simulink model "Radial_Grid"  (R2024a)
settings: Solver=VariableStepAuto  StartTime=0.0  StopTime=1  RelTol=1e-3
undefined symbols (not defined in the file): D1, Delta
libraries: spsThreePhaseBreakerLib x8, spsGroundLib x7, spsThreePhaseParallelRLCLoadLib x7, spsThreePhaseVIMeasurementLib x5, eeRmsMeasurement x2, spsDistributedParametersLineLib x1, spsPLL3phLib x1, spsThreePhaseSourceLib x1, spsThreePhaseTransformerInductanceMatrixTypeTwoWindingsLib x1, sps_lib x1
settings Model: Creator=NIHUB  LastModifiedBy=NIHUB

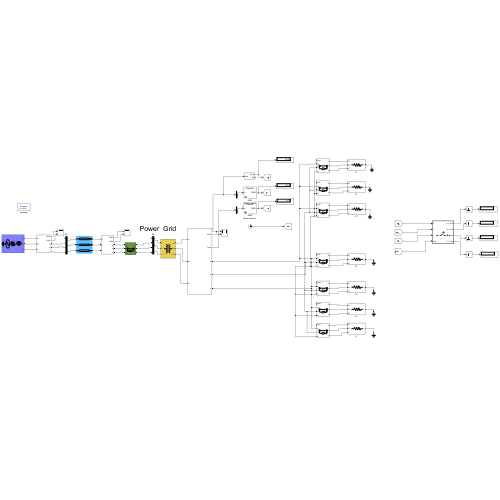
[thumbnail: Simulink's stored preview of the top-level diagram]
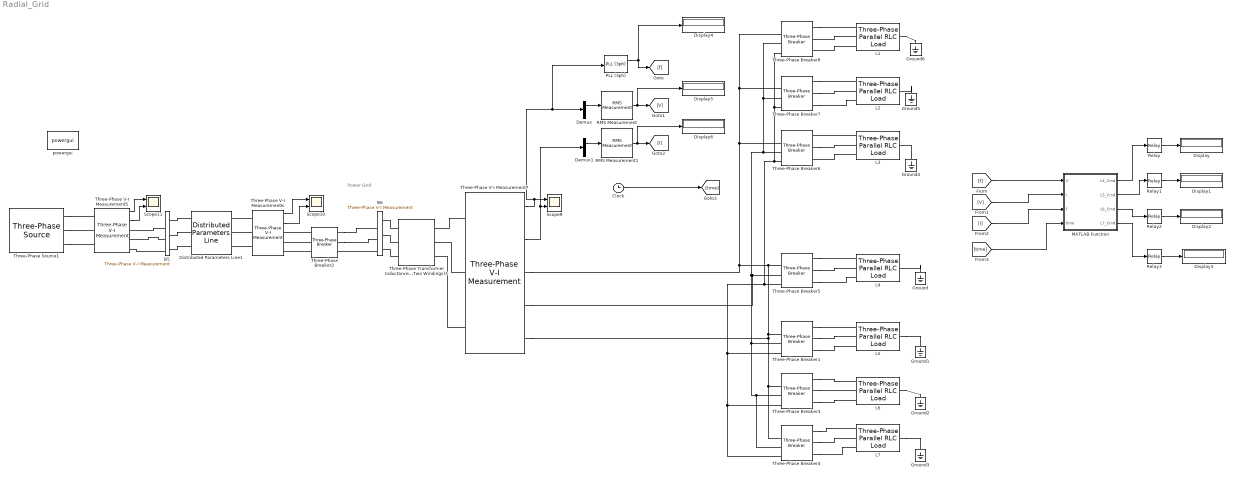
== system Radial_Grid ==
  note: Power Grid
  B5 : spsThreePhaseVIMeasurementLib/Three-Phase V-I Measurement  VoltageMeasurement=phase-to-ground  SetLabelV=off  LabelV=Vabc_B12  Vpu=off  VpuLL=off  CurrentMeasurement=no  SetLabelI=off  LabelI=A1  Ipu=off  Pbase=100e6  Vbase=25e3  OutputType=Magnitude  PhasorSimulation=off  PSBequivalent=0
  B6 : spsThreePhaseVIMeasurementLib/Three-Phase V-I Measurement  VoltageMeasurement=phase-to-phase  SetLabelV=off  LabelV=Vabc_B12  Vpu=off  VpuLL=off  CurrentMeasurement=no  SetLabelI=off  LabelI=A1  Ipu=off  Pbase=100e6  Vbase=440  OutputType=Magnitude  PhasorSimulation=off  PSBequivalent=0
  Clock : Clock
  Demux : Demux  Outputs=3
  Demux1 : Demux  Outputs=3
  Display{,1..6} (7 alike) : Display
  Distributed Parameters Line1 : spsDistributedParametersLineLib/Distributed Parameters Line  Phases=3  Length=100  Frequency=50  Resistance=[0.01273 0.3864]  Inductance="[0.9337e-3  4.1264e-3]"  Capacitance=[12.74e-9 7.751e-9]  x1=[-0.0006 -5.69435652062801e-12 3198.12006317178 -10428.926964129;-0.00055 -5.76202165425784e-12 3395.1058429697 -10367.660250018;-0.0005 -5.82763956903046e-12 3590.88535782781 -10302.709955587;-0.00045 -5.8911869512132e-12 3785.38904821671 -10234.0991573664;-0.0004 -5.95264122272375e-12 3978.54780790135 -10161.852232446;-0.00035 -6.01198054915207e-12 4170.29300849417 -10085.9948498143;-0.0003 -6.06918384751803e-12 4360.55652383841 -10006.5539612381;-0.00025 -6.1242307937621e-12 4549.27075421304 -9923.55779168682;-0.0002 -6.1771018299664e-12 4736.36865035058 -9837.03582930438;-0.00015 -6.22777817130351e-12 4921.78373725944 -9747.018814932;-0.0001 -6.27624181271066e-12 5105.4501378421 -9653.53873118626;-5e-05 -6.32247553528681e-12 5287.30259630099 -9556.62879109579]  x2=[-0.0006 9.88072191954148e-12 2341.94542948647 -8036.57356519092;-0.00055 3.91022286306686e-12 2519.49823419962 -8019.58597186587;-0.0005 -2.06166547697203e-12 2696.15587318705 -7999.74905783124;-0.00045 -8.03282131708381e-12 2871.8555808308 -7977.0698710481;-0.0004 -1.40011231340308e-11 3046.53493186135 -7951.55646932354;-0.00035 -1.99644504185964e-11 3220.13186353705 -7923.2179174477;-0.0003 -2.59206844289913e-11 3392.58469769468 -7892.06428397313;-0.00025 -3.18677089436329e-11 3563.83216266341 -7858.10663763746;-0.0002 -3.78034110130288e-11 3733.81341503435 -7821.35704343074;-0.00015 -4.37256817104971e-11 3902.46806127792 -7781.82855830881;-0.0001 -4.96324168814587e-11 4069.73617920138 -7739.5352265542;-5e-05 -5.55215178910329e-11 4235.5583392389 -7694.4920747863]  x3=[-0.0006 1.90091766669321e-12 37.8763934062412 29.3478799697958;-0.00055 1.89376898505282e-12 38.1331821574926 30.7493103327158;-0.0005 1.88594745630945e-12 38.376422370699 32.139815612091;-0.00045 1.87745585941501e-12 38.606027623771 33.5189017680168;-0.0004 1.86829721139346e-12 38.8219163390555 34.8860788177486;-0.00035 1.85847476626881e-12 39.0240118123198 36.2408610097907;-0.0003 1.84799201390905e-12 39.2122422400046 37.5827669964811;-0.00025 1.83685267878618e-12 39.3865407447353 38.9113200050124;-0.0002 1.82506071865293e-12 39.546845399083 40.2260480068268;-0.00015 1.81262032313659e-12 39.6930992475674 41.5264838853255;-0.0001 1.79953591225044e-12 39.8252503268925 42.8121656018329;-5e-05 1.78581213482337e-12 39.9432516844091 44.0826363597572]  x4=[-0.0006 -1.86563145591836e-12 -22.2642144665342 -98.2708522257449;-0.00055 -1.86603152740087e-12 -21.1164830183401 -99.4675733684154;-0.0005 -1.86576860676702e-12 -19.9612489842783 -100.628954155895;-0.00045 -1.86484278743127e-12 -18.7989228135002 -101.754581955119;-0.0004 -1.86325439833281e-12 -17.6299174749598 -102.844056835891;-0.00035 -1.86100400381873e-12 -16.4546483106874 -103.896991712974;-0.0003 -1.85809240344349e-12 -15.2735328882211 -104.913012483619;-0.00025 -1.85452063168482e-12 -14.0869908522462 -105.891758160483;-0.0002 -1.85028995757624e-12 -12.8954437754984 -106.83288099989;-0.00015 -1.84540188425611e-12 -11.6993150089804 -107.736046625375;-0.0001 -1.8398581484336e-12 -10.4990295315473 -108.600934146491;-5e-05 -1.83366071977165e-12 -9.29501379891409 -109.427236272822]  x5=0.000565541566995743  V1=[0 0 0 2.339e-09 6.456e+04 6.456e+04;0 0 0 314.2 314.2 314.2;1.571 1.571 1.571 -0.9334 0.4129 -1.158]  V2=[0 0 0 9.955e-09 6.494e+04 6.494e+04;0 0 0 314.2 314.2 314.2;1.571 1.571 1.571 -1.047 0.4126 -1.158]  I1=[0 0 0 5.638e-11 239 239;0 0 0 314.2 314.2 314.2;1.571 1.571 1.571 -2.312 0.3045 -1.266]  I2=[0 0 0 5.238e-11 239.1 239.1;0 0 0 314.2 314.2 314.2;1.571 1.571 1.571 0.5382 0.4125 -1.158]  nHarmo=2  Measurements=None  Decoupling=off  VsMag0=0  VrMag0=0  VsAngle0=0  VrAngle0=0  IsMag0=0  IrMag0=0  IsAngle0=0  IrAngle0=0
      settings: LibrarySourceBlock=sps_lib/Power Grid Elements/Distributed Parameters Line
  Ground{,1..6} (7 alike) : spsGroundLib/Ground  LConnTagsString=a
  L1 : spsThreePhaseParallelRLCLoadLib/Three-Phase Parallel RLC Load  LConnTagsString=A|B|C  RConnTagsString=N  Configuration=Y (neutral)  NominalVoltage=400  Vabc=[1e3 1e3 1e3]  Vabcp=[1e3 1e3 1e3]  NominalFrequency=50  UnbalancedPower=off  ActivePower=300e3  InductivePower=0  CapacitivePower=0  Pabc=[10e3 9e3 11e3]  QLabc=[100 90 110]  QCabc=[100 90 110]  Pabcp=[10e3 9e3 11e3]  QLabcp=[100 90 110]  QCabcp=[100 90 110]  Measurements=Branch voltages and currents  LoadType=constant PQ
  L2 : spsThreePhaseParallelRLCLoadLib/Three-Phase Parallel RLC Load  LConnTagsString=A|B|C  RConnTagsString=N  Configuration=Y (neutral)  NominalVoltage=400  Vabc=[1e3 1e3 1e3]  Vabcp=[1e3 1e3 1e3]  NominalFrequency=50  UnbalancedPower=off  ActivePower=250e3  InductivePower=0  CapacitivePower=0  Pabc=[10e3 9e3 11e3]  QLabc=[100 90 110]  QCabc=[100 90 110]  Pabcp=[10e3 9e3 11e3]  QLabcp=[100 90 110]  QCabcp=[100 90 110]  Measurements=Branch voltages and currents  LoadType=constant PQ
  L3 : spsThreePhaseParallelRLCLoadLib/Three-Phase Parallel RLC Load  LConnTagsString=A|B|C  RConnTagsString=N  Configuration=Y (neutral)  NominalVoltage=400  Vabc=[1e3 1e3 1e3]  Vabcp=[1e3 1e3 1e3]  NominalFrequency=50  UnbalancedPower=off  ActivePower=200e3  InductivePower=0  CapacitivePower=0  Pabc=[10e3 9e3 11e3]  QLabc=[100 90 110]  QCabc=[100 90 110]  Pabcp=[10e3 9e3 11e3]  QLabcp=[100 90 110]  QCabcp=[100 90 110]  Measurements=Branch voltages and currents  LoadType=constant PQ
  L4 : spsThreePhaseParallelRLCLoadLib/Three-Phase Parallel RLC Load  LConnTagsString=A|B|C  RConnTagsString=N  Configuration=Y (neutral)  NominalVoltage=400  Vabc=[1e3 1e3 1e3]  Vabcp=[1e3 1e3 1e3]  NominalFrequency=50  UnbalancedPower=off  ActivePower=180e3  InductivePower=0  CapacitivePower=0  Pabc=[10e3 9e3 11e3]  QLabc=[100 90 110]  QCabc=[100 90 110]  Pabcp=[10e3 9e3 11e3]  QLabcp=[100 90 110]  QCabcp=[100 90 110]  Measurements=Branch voltages and currents  LoadType=constant PQ
  L5 : spsThreePhaseParallelRLCLoadLib/Three-Phase Parallel RLC Load  LConnTagsString=A|B|C  RConnTagsString=N  Configuration=Y (neutral)  NominalVoltage=400  Vabc=[1e3 1e3 1e3]  Vabcp=[1e3 1e3 1e3]  NominalFrequency=50  UnbalancedPower=off  ActivePower=120e3  InductivePower=0  CapacitivePower=0  Pabc=[10e3 9e3 11e3]  QLabc=[100 90 110]  QCabc=[100 90 110]  Pabcp=[10e3 9e3 11e3]  QLabcp=[100 90 110]  QCabcp=[100 90 110]  Measurements=Branch voltages and currents  LoadType=constant PQ
  L6 : spsThreePhaseParallelRLCLoadLib/Three-Phase Parallel RLC Load  LConnTagsString=A|B|C  RConnTagsString=N  Configuration=Y (neutral)  NominalVoltage=400  Vabc=[1e3 1e3 1e3]  Vabcp=[1e3 1e3 1e3]  NominalFrequency=50  UnbalancedPower=off  ActivePower=100e3  InductivePower=0  CapacitivePower=0  Pabc=[10e3 9e3 11e3]  QLabc=[100 90 110]  QCabc=[100 90 110]  Pabcp=[10e3 9e3 11e3]  QLabcp=[100 90 110]  QCabcp=[100 90 110]  Measurements=Branch voltages and currents  LoadType=constant PQ
  L7 : spsThreePhaseParallelRLCLoadLib/Three-Phase Parallel RLC Load  LConnTagsString=A|B|C  RConnTagsString=N  Configuration=Y (neutral)  NominalVoltage=400  Vabc=[1e3 1e3 1e3]  Vabcp=[1e3 1e3 1e3]  NominalFrequency=50  UnbalancedPower=off  ActivePower=150e3  InductivePower=0  CapacitivePower=0  Pabc=[10e3 9e3 11e3]  QLabc=[100 90 110]  QCabc=[100 90 110]  Pabcp=[10e3 9e3 11e3]  QLabcp=[100 90 110]  QCabcp=[100 90 110]  Measurements=Branch voltages and currents  LoadType=constant PQ
  MATLAB Function : MATLAB Function  TreatAsAtomicUnit=on
  PLL (3ph) : spsPLL3phLib/PLL (3ph)  Fmin=45  Par_Init=[0, 50]  ParK=[180, 3200, 1]  TcD=1e-4  MaxRateChangeFreq=12  FilterCutOffFreq=25  Ts=50e-6  AGC=on
  RMS Measurement : eeRmsMeasurement/RMS Measurement  LabelModeActiveChoice=Total  F=50  SpecifyHarmonics=off  K=[0 1 2]  Ts=50e-6
      settings: LibrarySourceBlock=|
      | ee_sl_lib/Measurements/RMS
      | Measurement
  RMS Measurement1 : eeRmsMeasurement/RMS Measurement  LabelModeActiveChoice=Total  F=50  SpecifyHarmonics=off  K=[0 1 2]  Ts=50e-6
      settings: LibrarySourceBlock=|
      | ee_sl_lib/Measurements/RMS
      | Measurement
  Relay{,1..3} (4 alike) : Relay
  Scope10 : Scope  NumInputPorts=2
  Scope11 : Scope  NumInputPorts=2
  Scope9 : Scope  NumInputPorts=2
  Three-Phase V-I Measurement5 : spsThreePhaseVIMeasurementLib/Three-Phase V-I Measurement  VoltageMeasurement=phase-to-ground  SetLabelV=off  LabelV=Vabc  Vpu=off  VpuLL=off  CurrentMeasurement=yes  SetLabelI=off  LabelI=Iabc  Ipu=off  Pbase=100e6  Vbase=500e3  OutputType=Complex  PhasorSimulation=off  PSBequivalent=0
  Three-Phase V-I Measurement6 : spsThreePhaseVIMeasurementLib/Three-Phase V-I Measurement  VoltageMeasurement=phase-to-ground  SetLabelV=off  LabelV=Vabc  Vpu=off  VpuLL=off  CurrentMeasurement=yes  SetLabelI=off  LabelI=Iabc  Ipu=off  Pbase=100e6  Vbase=500e3  OutputType=Complex  PhasorSimulation=off  PSBequivalent=0
  Three-Phase V-I Measurement7 : spsThreePhaseVIMeasurementLib/Three-Phase V-I Measurement  VoltageMeasurement=phase-to-phase  SetLabelV=off  LabelV=Vabc_b1  Vpu=off  VpuLL=off  CurrentMeasurement=yes  SetLabelI=off  LabelI=Iabc_b1  Ipu=off  Pbase=100e6  Vbase=500e3  OutputType=Complex  PhasorSimulation=off  PSBequivalent=0
  Three-Phase Breaker{1,3..8} (7 alike) : spsThreePhaseBreakerLib/Three-Phase Breaker  InitialState=closed  SwitchA=off  SwitchB=off  SwitchC=off  SwitchTimes="[1/60  5/60]"  External=on  BreakerResistance=0.01  SnubberResistance=1e6  SnubberCapacitance=inf  Measurements=None
  Three-Phase Breaker2 : spsThreePhaseBreakerLib/Three-Phase Breaker  InitialState=closed  SwitchA=off  SwitchB=off  SwitchC=off  SwitchTimes="[1/50  20/50]"  External=off  BreakerResistance=0.001  SnubberResistance=1e6  SnubberCapacitance=inf  Measurements=None
  Three-Phase Source1 : spsThreePhaseSourceLib/Three-Phase Source  InternalConnection=Yg  VoltagePhases=off  Voltage=11000  PhaseAngle=0  Voltage_phases=[25e3 25e3 25e3]/sqrt(3)  PhaseAngles_phases=[0 -120 +120]  Frequency=60  NonIdealSource=on  SpecifyImpedance=on  Resistance=0.8929  Inductance=16.58e-3  ShortCircuitLevel=100e6  BaseVoltage=11000  XRratio=7  BusType=swing  Pref=0  Qref=0  Prefabc=[10e3, 10e3, 10e3]  Qrefabc=[0, 0, 0]  Qmin=-inf  Qmax=inf
  Three-Phase Transformer Inductance Matrix Type (Two Windings)3 : spsThreePhaseTransformerInductanceMatrixTypeTwoWindingsLib/Three-Phase Transformer Inductance Matrix Type (Two Windings)  CoreType=Three-limb or five-limb core  Winding1Connection=Delta (D1)  Winding2Connection=Delta (D1)  AutoTransformer=off  Measurements=None  NominalPower=[100e3 50]  VLLnom=[11000 400]  WindingResistances=[0.01 0.01]  NoLoadIexcPos=2  NoLoadPlossPos=1000  ShortCircuitReactancePos=0.06  ShortCircuitReactancePosAuto=0.06  NoLoadIexcZero=100  NoLoadPlossZero=1500  ShortCircuitReactanceZero=0.03  ShortCircuitReactanceZeroAuto=0.03
      settings: LibrarySourceBlock=|
      | sps_lib/Power Grid Elements/Three-Phase Transformer
      | Inductance Matrix Type
      | (Two Windings)
  powergui : sps_lib/powergui  Priority=1  SimulationMode=Discrete  SampleTime=50e-6  frequency=60  Iterations=50  frequencyindice=0  Pbase=100e6  ErrMax=1e-4  UnitsV=kV  UnitsW=MW  buscounter=0  FunctionMessages=off  echomessages=off  EnableUseOfTLC=off  CurrentSourceSwitches=off  DisableSnubberDevices=off  DisableRonSwitches=off  DisableVfSwitches=off  DisplayEquations=off  AutomaticDiscreteSolvers=off  SolverType=Tustin  Interpol=off  ExternalGateDelay=off  methode=off  Ts=0  x0status=blocks  SPID=off  SwTol=0  HookPort=off  NonlinearTolerance=1e-4  nMaxIteration=100  ContinueOnMaxIteration=off  RestoreLinks=warning  ResistiveCurrentMeasurement=off  Frange=[0:2:500]  Ylog=off  Xlog=on  ShowGrid=off  save=off  variable=ZData  structure=0  ZoomFFT=off  StartTime=0.0  cycles=1  DisplayStyle=1  fundamental=60  FreqAxis=off  MaxFrequency=1000  frequencyindicesteady=1  RmsSteady=1  display=off
  wires:
  [f] -> MATLAB Function/1(V)
  [V] -> MATLAB Function/2(I)
  [I] -> MATLAB Function/3(f)
  [time] -> MATLAB Function/4(time)
  MATLAB Function/1(L4_Cmd) -> Relay/1
  MATLAB Function/2(L5_Cmd) -> Relay1/1
  MATLAB Function/3(L6_Cmd) -> Relay2/1
  MATLAB Function/4(L7_Cmd) -> Relay3/1
  Relay3/1 -> Display3/1
  Relay2/1 -> Display2/1
  Relay1/1 -> Display1/1
  Relay/1 -> Display/1
  Demux1/1 -> RMS Measurement1/1
  RMS Measurement/1 -> Display5/1, [V]
  RMS Measurement1/1 -> Display6/1, [I]
  Three-Phase V-I Measurement6/1 -> Scope10/1
  Three-Phase V-I Measurement5/2 -> Scope11/2
  Three-Phase V-I Measurement5/1 -> Scope11/1
  Three-Phase V-I Measurement7/2 -> Demux1/1, Scope9/2
  Three-Phase V-I Measurement6/2 -> Scope10/2
  Demux/1 -> RMS Measurement/1
  PLL (3ph)/1 -> Display4/1, [f]
  Three-Phase V-I Measurement7/1 -> PLL (3ph)/1, Demux/1, Scope9/1
  Clock/1 -> [time]
  connections:
  Ground/LConn1 -- L4/RConn1
  Ground5/LConn1 -- L2/RConn1
  L1/RConn1 -- Ground6/LConn1
  Ground4/LConn1 -- L3/RConn1
  L5/RConn1 -- Ground1/LConn1
  L6/RConn1 -- Ground2/LConn1
  L7/RConn1 -- Ground3/LConn1
  Three-Phase Breaker1/RConn1 -- L5/LConn1
  Three-Phase Breaker1/RConn2 -- L5/LConn2
  Three-Phase Breaker1/RConn3 -- L5/LConn3
  Three-Phase Breaker3/RConn1 -- L6/LConn1
  Three-Phase Breaker3/RConn2 -- L6/LConn2
  Three-Phase Breaker3/RConn3 -- L6/LConn3
  Three-Phase Breaker4/RConn1 -- L7/LConn1
  Three-Phase Breaker4/RConn2 -- L7/LConn2
  Three-Phase Breaker4/RConn3 -- L7/LConn3
  Three-Phase Breaker5/RConn1 -- L4/LConn1
  Three-Phase Breaker5/RConn2 -- L4/LConn2
  Three-Phase Breaker5/RConn3 -- L4/LConn3
  Three-Phase Breaker5/LConn1 -- Three-Phase Breaker4/LConn1 -- Three-Phase Breaker3/LConn1 -- Three-Phase V-I Measurement7/RConn3 -- Three-Phase Breaker1/LConn1 -- Three-Phase Breaker8/LConn1 -- Three-Phase Breaker7/LConn1 -- Three-Phase Breaker6/LConn1 -- Three-Phase V-I Measurement7/RConn1
  Three-Phase Breaker4/LConn2 -- Three-Phase Breaker3/LConn2 -- Three-Phase Breaker1/LConn2 -- Three-Phase Breaker8/LConn2 -- Three-Phase Breaker7/LConn2 -- Three-Phase Breaker6/LConn2 -- Three-Phase V-I Measurement7/RConn2 -- Three-Phase Breaker5/LConn2
  Three-Phase Breaker1/LConn3 -- Three-Phase Breaker4/LConn3 -- Three-Phase Breaker3/LConn3 -- Three-Phase Breaker8/LConn3 -- Three-Phase Breaker7/LConn3 -- Three-Phase Breaker6/LConn3 -- Three-Phase Breaker5/LConn3
  Three-Phase Breaker8/RConn1 -- L1/LConn1
  L1/LConn2 -- Three-Phase Breaker8/RConn2
  L1/LConn3 -- Three-Phase Breaker8/RConn3
  Three-Phase Breaker7/RConn1 -- L2/LConn1
  Three-Phase Breaker7/RConn2 -- L2/LConn2
  Three-Phase Breaker7/RConn3 -- L2/LConn3
  L3/LConn1 -- Three-Phase Breaker6/RConn1
  Three-Phase Breaker6/RConn2 -- L3/LConn2
  L3/LConn3 -- Three-Phase Breaker6/RConn3
  B5/RConn1 -- Three-Phase V-I Measurement5/RConn1
  Three-Phase V-I Measurement7/LConn2 -- Three-Phase Transformer Inductance Matrix Type (Two Windings)3/RConn2
  Three-Phase V-I Measurement6/LConn1 -- Distributed Parameters Line1/RConn1
  Three-Phase Breaker2/RConn1 -- Three-Phase V-I Measurement6/RConn1
  Three-Phase Breaker2/RConn2 -- Three-Phase V-I Measurement6/RConn2
  Three-Phase Transformer Inductance Matrix Type (Two Windings)3/LConn3 -- B6/LConn3
  Three-Phase Transformer Inductance Matrix Type (Two Windings)3/LConn2 -- B6/LConn2
  Three-Phase V-I Measurement6/LConn3 -- Distributed Parameters Line1/RConn3
  Three-Phase Breaker2/LConn1 -- B6/RConn1
  Distributed Parameters Line1/LConn1 -- B5/LConn1
  Distributed Parameters Line1/LConn2 -- B5/LConn2
  Three-Phase V-I Measurement7/LConn1 -- Three-Phase Transformer Inductance Matrix Type (Two Windings)3/RConn1
  Three-Phase Source1/RConn1 -- Three-Phase V-I Measurement5/LConn1
  B5/RConn2 -- Three-Phase V-I Measurement5/RConn2
  Three-Phase Source1/RConn2 -- Three-Phase V-I Measurement5/LConn2
  Three-Phase V-I Measurement6/LConn2 -- Distributed Parameters Line1/RConn2
  Three-Phase Source1/RConn3 -- Three-Phase V-I Measurement5/LConn3
  Distributed Parameters Line1/LConn3 -- B5/LConn3
  Three-Phase Transformer Inductance Matrix Type (Two Windings)3/LConn1 -- B6/LConn1
  Three-Phase V-I Measurement7/LConn3 -- Three-Phase Transformer Inductance Matrix Type (Two Windings)3/RConn3
  Three-Phase Breaker2/LConn2 -- B6/RConn2
  B5/RConn3 -- Three-Phase V-I Measurement5/RConn3
  B6/RConn3 -- Three-Phase Breaker2/LConn3
  Three-Phase Breaker2/RConn3 -- Three-Phase V-I Measurement6/RConn3

== matlab function Radial_Grid/MATLAB Function ==
  data: V input; L4_Cmd output; I input; f input; time input; L5_Cmd output; L6_Cmd output; L7_Cmd output
function [L4_Cmd, L5_Cmd, L6_Cmd, L7_Cmd] = controlAlgorithm(V, I, f, time)
% controlAlgorithm: Main control logic for the load shedding system.
% This function is a single block that handles all calculations,
% decision-making, and control outputs for the microgrid.
%
% Inputs:
% V: Measured voltage (Volts)
% I: Measured current (Amperes)
% f: Measured frequency (Hertz)
% time: Simulation time from the Simulink Clock block (seconds)
%
% Outputs:
% L4_Cmd, L5_Cmd, L6_Cmd, L7_Cmd: Binary control signals (1 = ON, 0 = OFF)

% --- 1. PERSISTENT STATE VARIABLES ---
% Persistent variables retain their values between function calls. This is
% crucial for maintaining the state of the relays and the power history.
persistent P_history;
persistent L4_state L5_state L6_state L7_state;

% Initialize state variables on the first call
if isempty(L4_state)
    L4_state = 1; % 1 = ON (connected), 0 = OFF (shed)
    L5_state = 1;
    L6_state = 1;
    L7_state = 1;
    P_history = zeros(1, 60); % A buffer to store 60 samples for the 1-second moving average
end

% --- 2. POWER CALCULATION ---
% Calculate the instantaneous power and the moving average power.
% The power factor (cos phi) is assumed to be 0.9.
P_inst = V * I * 0.9;
% Check for negative power values (e.g., from sensor noise) and set to 0
if P_inst < 0
    P_inst = 0;
end

% Update the moving average history buffer.
% This shifts the history and adds the new sample.
P_history = [P_history(2:end), P_inst];
P_avg = mean(P_history);

% --- 3. TIME-BASED PRIORITY WEIGHTS ---
% Define the fixed and dynamic weights for all loads based on time.
% This section implements the dynamic prioritization logic.
L1_weight = 0.95; % Hospital (Critical)
L2_weight = 0.90; % Water Treatment Plant (Critical)
L3_weight = 0.85; % Government Secretariat (Critical)
L5_weight = 0.40; % Secondary School (Semi-Priority)
L6_weight = 0.20; % Street Lighting (Less-Priority)

% Adjust L4 (Mall) and L7 (Residential) weights based on time of day.
% The simulation time is treated as hours for simplicity.
if (time >= 6 && time < 14) % Morning (6 AM - 2 PM)
    L4_weight = 0.50;
    L7_weight = 0.10;
elseif (time >= 18 || time < 6) % Evening/Night (6 PM - 6 AM)
    L4_weight = 0.10;
    L7_weight = 0.50;
else % Afternoon (2 PM - 6 PM)
    L4_weight = 0.50;
    L7_weight = 0.10;
end

% --- 4. OVERLOAD DETECTION AND SHEDDING ---
% Check for any overload condition based on the defined thresholds.
% If an overload is detected, initiate the shedding sequence.
if (P_avg > 1250 || P_inst > 1300 || f < 59 || V < 360)
    
    % Create a struct array to manage non-critical loads and their properties.
    % This makes sorting and iteration much cleaner.
    loads_to_shed = [
        struct('id', 'L7', 'weight', L7_weight, 'power', 150000, 'state', L7_state);
        struct('id', 'L6', 'weight', L6_weight, 'power', 100000, 'state', L6_state);
        struct('id', 'L5', 'weight', L5_weight, 'power', 120000, 'state', L5_state);
        struct('id', 'L4', 'weight', L4_weight, 'power', 180000, 'state', L4_state)
    ];
    
    % Sort the loads by ascending weight (lowest priority first).
    [~, sorted_indices] = sort([loads_to_shed.weight]);
    sorted_loads = loads_to_shed(sorted_indices);
    
    % Iterate through the sorted loads and shed them one by one
    % until the power is below the threshold.
    total_shed_power = 0; % Track how much power we've shed
    for i = 1:length(sorted_loads)
        current_load = sorted_loads(i);
        if current_load.state == 1 % Check if the load is currently connected
            total_shed_power = total_shed_power + current_load.power;
            
            % Update the persistent state for the load being shed.
            switch current_load.id
                case 'L4', L4_state = 0;
                case 'L5', L5_state = 0;
                case 'L6', L6_state = 0;
                case 'L7', L7_state = 0;
            end
            
            % Check if the power is now within a safe range after shedding.
            % The (P_inst - total_shed_power) is a simple estimate.
            if (P_inst - total_shed_power) <= 1250
                break; % Stop shedding once power is safe
            end
        end
    end
    
% --- 5. LOAD RESTORATION ---
% Check for stable conditions to restore previously shed loads.
% The threshold for restoration is stricter to prevent cycling (chattering).
elseif (P_inst <= 1300 && f >= 59.5 && V >= 380)
    % A simple restoration logic: reconnect all loads if the system is stable.
    L4_state = 1;
    L5_state = 1;
    L6_state = 1;
    L7_state = 1;
end

% --- 6. ASSIGN OUTPUTS ---
% Assign the final persistent state of each load to the output variables.
L4_Cmd = L4_state;
L5_Cmd = L5_state;
L6_Cmd = L6_state;
L7_Cmd = L7_state;

end
